simulink model "sfMotorFixedDirect"  (R2025b)
settings: Solver=VariableStepAuto  StartTime=0.0  StopTime=10.0  RelTol=1e-3
settings Model: Creator=The MathWorks, Inc.  LastModifiedBy=The MathWorks, Inc.

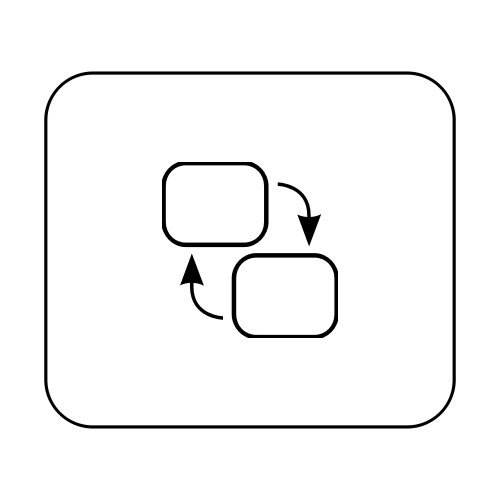
[thumbnail: Simulink's stored preview of the top-level diagram]
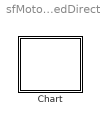
== system sfMotorFixedDirect ==
  Chart : Stateflow chart  TreatAsAtomicUnit=on

== stateflow chart sfMotorFixedDirect/Chart ==
  state Motor [parallel]
    settings: executionOrder=1
    state Off
    state On
    state Idle
    (default) -> Motor.Off
    Motor.Off -> Motor.On : {send(cooling_on,Vent)
        | send(cooling_on,Fan)}
    (junction 28) -> Motor.Off
    Motor.On -> Idle
    Idle -> (junction 28) : {send(cooling_off,Vent)
        | send(cooling_off,Fan)}
  state Vent [parallel]
    settings: executionOrder=2
    state Low
    state High
    (default) -> Low
    Low -> High : cooling_on
    High -> Low : cooling_off
  state Fan [parallel]
    settings: executionOrder=3
    state Off
    state On
    (default) -> Fan.Off
    Fan.Off -> Fan.On : cooling_on
    Fan.On -> Fan.Off : cooling_off
  events: cooling_off local FUNCTION_CALL_EVENT; cooling_on local FUNCTION_CALL_EVENT
